simulink model "rfid_tracking"  (R2026b)
settings: Solver=FixedStepDiscrete  StopTime=controlConfig.stopTime  FixedStep=controlConfig.dt
model workspace (MAT data in the model file):
  controlConfig.controllerConfig = controls.ControllerConfig
  controlConfig.controllerMode = 1
  controlConfig.output = '/Users/fcp/Desktop/Schoolwork/Controls/ControlsProject/matlab/output/tracking.csv'
  controlConfig.particles = 500
  controlConfig.plot = 1
  controlConfig.seed = 42
  controlConfig.sensorConfig = controls.RFIDConfig
  controlConfig.dt = 0.1
  controlConfig.stopTime = 20
  controlConfig.workspace = [0 10 0 10]
  controlConfig.requirements.positionRMSE = 0.5
  controlConfig.requirements.validTimeRate = 95
  controlConfig.requirements.recoveryTime = 3
  controlScenario : object (value not decoded)
settings Model: Creator=fcp  LastModifiedBy=fcp
settings DebuggingCC: AlgebraicLoopMsg=error

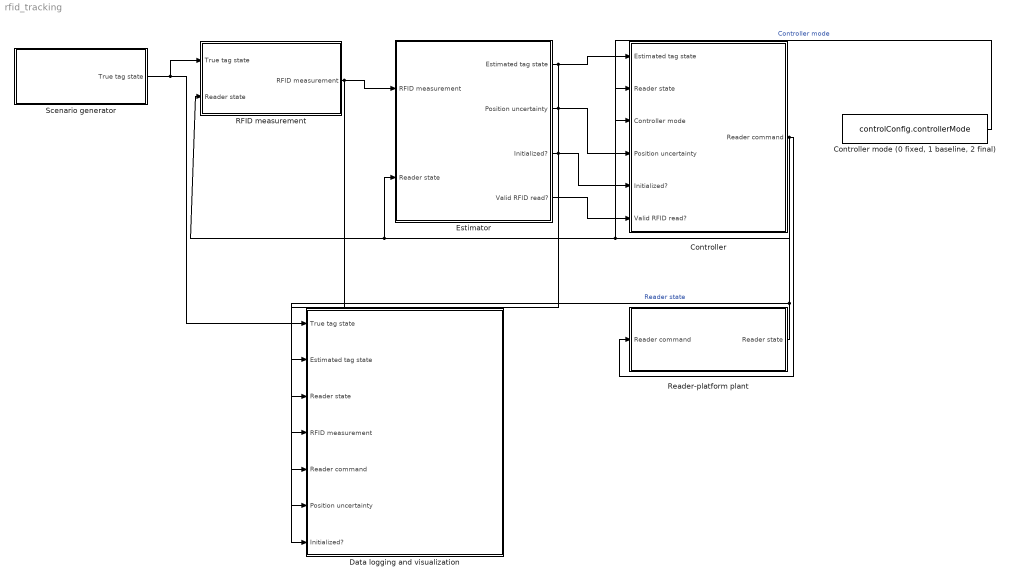
== system rfid_tracking ==
  Controller : Subsystem
  "Controller mode (0 fixed, 1 baseline, 2 final)" : Constant  Value=controlConfig.controllerMode
  Data logging and visualization : Subsystem
  Estimator : Subsystem
  RFID measurement : Subsystem
  Reader-platform plant : Subsystem
  Scenario generator : Subsystem
  wires:
  Scenario generator/1(True tag state) -> RFID measurement/1(True tag state), Data logging and visualization/1(True tag state)
  Reader-platform plant/1(Reader state) -> RFID measurement/2(Reader state), Estimator/2(Reader state), Controller/2(Reader state), Data logging and visualization/3(Reader state)  "Reader state"
  RFID measurement/1(RFID measurement) -> Estimator/1(RFID measurement), Data logging and visualization/4(RFID measurement)
  Estimator/1(Estimated tag state) -> Controller/1(Estimated tag state), Data logging and visualization/2(Estimated tag state)
  Estimator/2(Position uncertainty) -> Controller/4(Position uncertainty), Data logging and visualization/6(Position uncertainty)
  Estimator/3(Initialized?) -> Controller/5(Initialized?), Data logging and visualization/7(Initialized?)
  Estimator/4(Valid RFID read?) -> Controller/6(Valid RFID read?)
  "Controller mode (0 fixed, 1 baseline, 2 final)"/1 -> Controller/3(Controller mode)  "Controller mode"
  Controller/1(Reader command) -> Reader-platform plant/1(Reader command), Data logging and visualization/5(Reader command)

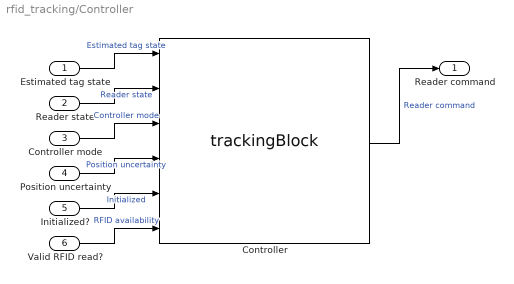
== system rfid_tracking/Controller ==
  Estimated tag state : Inport  PortDimensions=4
  Reader state : Inport  Port=2  PortDimensions=5
  Controller mode : Inport  Port=3  PortDimensions=1
  Position uncertainty : Inport  Port=4  PortDimensions=1
  Initialized? : Inport  Port=5  PortDimensions=1
  Valid RFID read? : Inport  Port=6  PortDimensions=1
  Controller : M-S-Function  FunctionName=trackingBlock  Parameters='controller','controlConfig','[]'
  Reader command : Outport
  wires:
  Estimated tag state/1 -> Controller/1  "Estimated tag state"
  Reader state/1 -> Controller/2  "Reader state"
  Controller mode/1 -> Controller/3  "Controller mode"
  Position uncertainty/1 -> Controller/4  "Position uncertainty"
  Initialized?/1 -> Controller/5  "Initialized"
  Valid RFID read?/1 -> Controller/6  "RFID availability"
  Controller/1 -> Reader command/1  "Reader command"

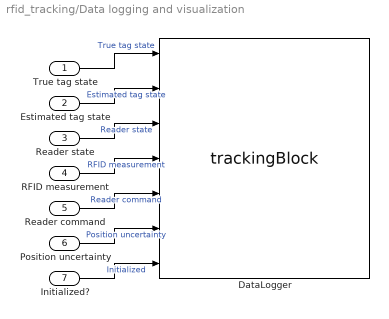
== system rfid_tracking/Data logging and visualization ==
  True tag state : Inport  PortDimensions=4
  Estimated tag state : Inport  Port=2  PortDimensions=4
  Reader state : Inport  Port=3  PortDimensions=5
  RFID measurement : Inport  Port=4  PortDimensions=6
  Reader command : Inport  Port=5  PortDimensions=2
  Position uncertainty : Inport  Port=6  PortDimensions=1
  Initialized? : Inport  Port=7  PortDimensions=1
  DataLogger : M-S-Function  FunctionName=trackingBlock  Parameters='logger','controlConfig','controlScenario.events'
  wires:
  True tag state/1 -> DataLogger/1  "True tag state"
  Estimated tag state/1 -> DataLogger/2  "Estimated tag state"
  Reader state/1 -> DataLogger/3  "Reader state"
  RFID measurement/1 -> DataLogger/4  "RFID measurement"
  Reader command/1 -> DataLogger/5  "Reader command"
  Position uncertainty/1 -> DataLogger/6  "Position uncertainty"
  Initialized?/1 -> DataLogger/7  "Initialized"

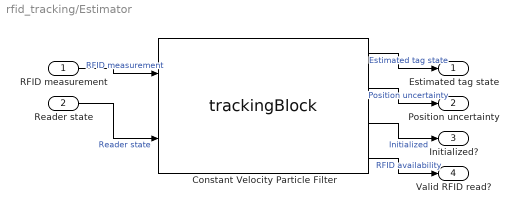
== system rfid_tracking/Estimator ==
  RFID measurement : Inport  PortDimensions=6
  Reader state : Inport  Port=2  PortDimensions=5
  Constant Velocity Particle Filter : M-S-Function  FunctionName=trackingBlock  Parameters='estimator','controlConfig','[]'
  Estimated tag state : Outport
  Position uncertainty : Outport  Port=2
  Initialized? : Outport  Port=3
  Valid RFID read? : Outport  Port=4
  wires:
  RFID measurement/1 -> Constant Velocity Particle Filter/1  "RFID measurement"
  Reader state/1 -> Constant Velocity Particle Filter/2  "Reader state"
  Constant Velocity Particle Filter/1 -> Estimated tag state/1  "Estimated tag state"
  Constant Velocity Particle Filter/2 -> Position uncertainty/1  "Position uncertainty"
  Constant Velocity Particle Filter/3 -> Initialized?/1  "Initialized"
  Constant Velocity Particle Filter/4 -> Valid RFID read?/1  "RFID availability"

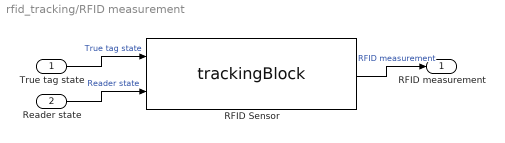
== system rfid_tracking/RFID measurement ==
  True tag state : Inport  PortDimensions=4
  Reader state : Inport  Port=2  PortDimensions=5
  RFID Sensor : M-S-Function  FunctionName=trackingBlock  Parameters='sensor','controlConfig','[]'
  RFID measurement : Outport
  wires:
  True tag state/1 -> RFID Sensor/1  "True tag state"
  Reader state/1 -> RFID Sensor/2  "Reader state"
  RFID Sensor/1 -> RFID measurement/1  "RFID measurement"

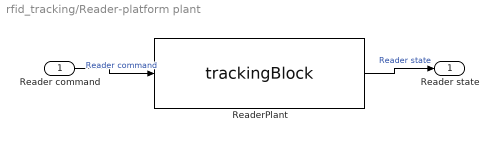
== system rfid_tracking/Reader-platform plant ==
  Reader command : Inport  PortDimensions=2
  ReaderPlant : M-S-Function  FunctionName=trackingBlock  Parameters='plant','controlConfig','[]'
  Reader state : Outport
  wires:
  Reader command/1 -> ReaderPlant/1  "Reader command"
  ReaderPlant/1 -> Reader state/1  "Reader state"

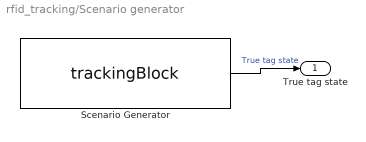
== system rfid_tracking/Scenario generator ==
  Scenario Generator : M-S-Function  FunctionName=trackingBlock  Parameters='scenario','controlScenario','[]'
  True tag state : Outport
  wires:
  Scenario Generator/1 -> True tag state/1  "True tag state"
